simulink model "AULA3"  (R2025b)
settings: Solver=VariableStepAuto  StartTime=0.0  StopTime=100  RelTol=1e-3
settings Model: Creator=RA00338338  LastModifiedBy=RA00338338

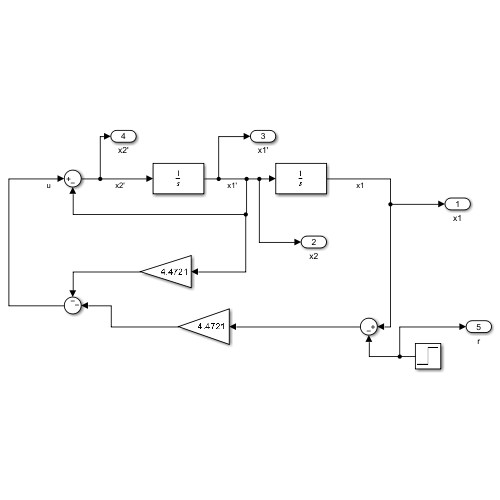
[thumbnail: Simulink's stored preview of the top-level diagram]
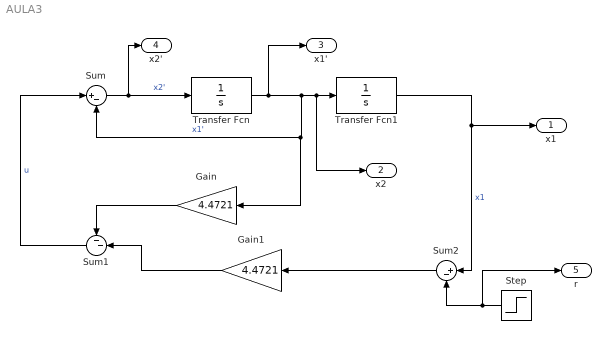
== system AULA3 ==
  Gain : Gain  Gain=4.4721
  Gain1 : Gain  Gain=4.4721
  Step : Step  Time=20  After=3  SampleTime=0
  Sum : Sum  Inputs=|+-
  Sum1 : Sum  Inputs=--|
  Sum2 : Sum  Inputs=|+-
  Transfer Fcn : TransferFcn  Denominator=[1 0]
  Transfer Fcn1 : TransferFcn  Denominator=[1 0]
  x1 : Outport
  x2 : Outport  Port=2
  x1' : Outport  Port=3
  x2' : Outport  Port=4
  r : Outport  Port=5
  wires:
  Sum/1 -> x2'/1, Transfer Fcn/1  "x2'"
  Transfer Fcn/1 -> x1'/1, Gain/1, Sum/2, x2/1, Transfer Fcn1/1  "x1'"
  Sum1/1 -> Sum/1  "u"
  Transfer Fcn1/1 -> x1/1, Sum2/1  "x1"
  Gain/1 -> Sum1/1
  Gain1/1 -> Sum1/2
  Sum2/1 -> Gain1/1
  Step/1 -> r/1, Sum2/2
